simulink library "Linkage"  (R2025b)
settings: Solver=VariableStepAuto  StartTime=0.0  StopTime=10.0  RelTol=1e-3
undefined symbols (not defined in the file): Axle1D, AxleIn, Chassis, Init, RaceFix, RaceSpin, Vehicle, Visual, X, Y, Z
libraries: sm_lib x940, nesl_utility x136, fl_lib x6, Linkage_Systems x2, SteeringWheel x2, Linkage_Decoupled x2, AntiRollBar_Systems x1, Steer_Rack_None x1, Steer_Rack_WheelDrivenRack1UJoint x1
(part 25 of 25)

== system Linkage/Susp/Linkage Decoupled/Steer/Wheel Driven Rack 1UJoint/Driver/Human/Leg L/Toe L ==
  ReferenceFrame : sm_lib/Frames and Transforms/Reference Frame
  Solid : sm_lib/Body Elements/File Solid  ExtGeomFileName=Human_toe_L.STEP  UnitType=FromFile  ExtGeomFileUnits=m  StepReaderType=HEX  ExportConvexHullGeometry=off  InertiaType=CalculateFromGeometry  BasedOnType=Density  Density=rho_human  DensityUnits=kg/m^3  Mass=0  MassUnits=kg  CenterOfMass=[0 0 0]  CenterOfMassUnits=mm  MomentsOfInertia=[1 1 1]  MomentsOfInertiaUnits=kg*mm^2  ProductsOfInertia=[0 0 0]  ProductsOfInertiaUnits=kg*mm^2  GraphicType=FromGeometry  MarkerShape=Sphere  MarkerSize=10  GraphicVisPropType=SimpleVisualProperties  GraphicDiffuseColor=clr_human  GraphicOpacity=opc_human  GraphicSpecularColor=[0.5 0.5 0.5 1.0]  GraphicAmbientColor=[0.15 0.15 0.15 1.0]  GraphicEmissiveColor=[0.0 0.0 0.0 1.0]  GraphicShininess=75  DoExposeReferenceFrame=on  SerializedFrames=<Frames/>
  Transform : sm_lib/Frames and Transforms/Rigid Transform  RotationMethod=ArbitraryAxis  FollAlignAxisA=+X  BaseAlignAxisA=+Y  FollAlignAxisB=+Y  BaseAlignAxisB=+Z  RotationStandardAxis=+Z  RotationAngle=0.087266462599702  RotationAngleUnits=rad  RotationArbitraryAxis=[1 -4.97119394825472e-15 -1.1612709063123e-14]  RotationSequenceAxes=FollowerAxes  RotationSequence=XYX  RotationSequenceAngles=[0 0 0]  RotationSequenceAnglesUnits=deg  RotationMatrix=[1 0 0; 0 1 0; 0 0 1]  Quaternion=[1 0 0 0]  TranslationMethod=Cartesian  TranslationCartesianOffset=[-1.46549439250521e-14 -82.7975674566105 4.68055928693002]  TranslationCartesianOffsetUnits=mm  TranslationStandardAxis=+Z  TranslationStandardOffset=0  TranslationStandardOffsetUnits=mm  TranslationROffset=0  TranslationROffsetUnits=m  TranslationThetaOffset=0  TranslationThetaOffsetUnits=deg  TranslationZOffset=0  TranslationZOffsetUnits=m
  F : PMIOPort  Side=Left
  connections:
  Transform/RConn1 -- F/RConn1
  Transform/LConn1 -- ReferenceFrame/RConn1 -- Solid/RConn1

== system Linkage/Susp/Linkage Decoupled/Steer/Wheel Driven Rack 1UJoint/Driver/Human/Leg R/Foot R ==
  ReferenceFrame : sm_lib/Frames and Transforms/Reference Frame
  Solid : sm_lib/Body Elements/File Solid  ExtGeomFileName=Human_foot_R.STEP  UnitType=FromFile  ExtGeomFileUnits=m  StepReaderType=HEX  ExportConvexHullGeometry=off  InertiaType=CalculateFromGeometry  BasedOnType=Density  Density=rho_human  DensityUnits=kg/m^3  Mass=0  MassUnits=kg  CenterOfMass=[0 0 0]  CenterOfMassUnits=mm  MomentsOfInertia=[1 1 1]  MomentsOfInertiaUnits=kg*mm^2  ProductsOfInertia=[0 0 0]  ProductsOfInertiaUnits=kg*mm^2  GraphicType=FromGeometry  MarkerShape=Sphere  MarkerSize=10  GraphicVisPropType=SimpleVisualProperties  GraphicDiffuseColor=clr_human  GraphicOpacity=opc_human  GraphicSpecularColor=[0.5 0.5 0.5 1.0]  GraphicAmbientColor=[0.15 0.15 0.15 1.0]  GraphicEmissiveColor=[0.0 0.0 0.0 1.0]  GraphicShininess=75  DoExposeReferenceFrame=on  SerializedFrames=<Frames/>
  Transform : sm_lib/Frames and Transforms/Rigid Transform  RotationMethod=ArbitraryAxis  FollAlignAxisA=+X  BaseAlignAxisA=+Y  FollAlignAxisB=+Y  BaseAlignAxisB=+Z  RotationStandardAxis=+Z  RotationAngle=0  RotationAngleUnits=rad  RotationArbitraryAxis=[0 0 0]  RotationSequenceAxes=FollowerAxes  RotationSequence=XYX  RotationSequenceAngles=[0 0 0]  RotationSequenceAnglesUnits=deg  RotationMatrix=[1 0 0; 0 1 0; 0 0 1]  Quaternion=[1 0 0 0]  TranslationMethod=Cartesian  TranslationCartesianOffset=[0 0 0]  TranslationCartesianOffsetUnits=mm  TranslationStandardAxis=+Z  TranslationStandardOffset=0  TranslationStandardOffsetUnits=mm  TranslationROffset=0  TranslationROffsetUnits=m  TranslationThetaOffset=0  TranslationThetaOffsetUnits=deg  TranslationZOffset=0  TranslationZOffsetUnits=m
  Transform1 : sm_lib/Frames and Transforms/Rigid Transform  RotationMethod=ArbitraryAxis  FollAlignAxisA=+X  BaseAlignAxisA=+Y  FollAlignAxisB=+Y  BaseAlignAxisB=+Z  RotationStandardAxis=+Z  RotationAngle=2.0943951023932  RotationAngleUnits=rad  RotationArbitraryAxis=[0.577350269189626 0.577350269189626 0.577350269189626]  RotationSequenceAxes=FollowerAxes  RotationSequence=XYX  RotationSequenceAngles=[0 0 0]  RotationSequenceAnglesUnits=deg  RotationMatrix=[1 0 0; 0 1 0; 0 0 1]  Quaternion=[1 0 0 0]  TranslationMethod=Cartesian  TranslationCartesianOffset=[-90.2524899999995 -95.0000000000001 -945.84775686]  TranslationCartesianOffsetUnits=mm  TranslationStandardAxis=+Z  TranslationStandardOffset=0  TranslationStandardOffsetUnits=mm  TranslationROffset=0  TranslationROffsetUnits=m  TranslationThetaOffset=0  TranslationThetaOffsetUnits=deg  TranslationZOffset=0  TranslationZOffsetUnits=m
  F1 : PMIOPort  Side=Left
  F : PMIOPort  Port=2  Side=Left
  connections:
  Transform1/RConn1 -- F1/RConn1
  Transform/RConn1 -- F/RConn1
  Transform1/LConn1 -- ReferenceFrame/RConn1 -- Solid/RConn1 -- Transform/LConn1

== system Linkage/Susp/Linkage Decoupled/Steer/Wheel Driven Rack 1UJoint/Driver/Human/Leg R/Leg Lower R ==
  ReferenceFrame : sm_lib/Frames and Transforms/Reference Frame
  Solid : sm_lib/Body Elements/File Solid  ExtGeomFileName=Human_leg_lower_R.STEP  UnitType=FromFile  ExtGeomFileUnits=m  StepReaderType=HEX  ExportConvexHullGeometry=off  InertiaType=CalculateFromGeometry  BasedOnType=Density  Density=rho_human  DensityUnits=kg/m^3  Mass=0  MassUnits=kg  CenterOfMass=[0 0 0]  CenterOfMassUnits=mm  MomentsOfInertia=[1 1 1]  MomentsOfInertiaUnits=kg*mm^2  ProductsOfInertia=[0 0 0]  ProductsOfInertiaUnits=kg*mm^2  GraphicType=FromGeometry  MarkerShape=Sphere  MarkerSize=10  GraphicVisPropType=SimpleVisualProperties  GraphicDiffuseColor=clr_human  GraphicOpacity=opc_human  GraphicSpecularColor=[0.5 0.5 0.5 1.0]  GraphicAmbientColor=[0.15 0.15 0.15 1.0]  GraphicEmissiveColor=[0.0 0.0 0.0 1.0]  GraphicShininess=75  DoExposeReferenceFrame=on  SerializedFrames=<Frames/>
  Transform : sm_lib/Frames and Transforms/Rigid Transform  RotationMethod=ArbitraryAxis  FollAlignAxisA=+X  BaseAlignAxisA=+Y  FollAlignAxisB=+Y  BaseAlignAxisB=+Z  RotationStandardAxis=+Z  RotationAngle=1.81417419955097  RotationAngleUnits=rad  RotationArbitraryAxis=[0.440666253836566 0.7820655378287 0.440666253836566]  RotationSequenceAxes=FollowerAxes  RotationSequence=XYX  RotationSequenceAngles=[0 0 0]  RotationSequenceAnglesUnits=deg  RotationMatrix=[1 0 0; 0 1 0; 0 0 1]  Quaternion=[1 0 0 0]  TranslationMethod=Cartesian  TranslationCartesianOffset=[-90.2524948099997 6.94251895000275 -465.147514340017]  TranslationCartesianOffsetUnits=mm  TranslationStandardAxis=+Z  TranslationStandardOffset=0  TranslationStandardOffsetUnits=mm  TranslationROffset=0  TranslationROffsetUnits=m  TranslationThetaOffset=0  TranslationThetaOffsetUnits=deg  TranslationZOffset=0  TranslationZOffsetUnits=m
  Transform1 : sm_lib/Frames and Transforms/Rigid Transform  RotationMethod=ArbitraryAxis  FollAlignAxisA=+X  BaseAlignAxisA=+Y  FollAlignAxisB=+Y  BaseAlignAxisB=+Z  RotationStandardAxis=+Z  RotationAngle=0.168839148981579  RotationAngleUnits=rad  RotationArbitraryAxis=[1 -1.13358649593422e-14 -2.20648188183204e-15]  RotationSequenceAxes=FollowerAxes  RotationSequence=XYX  RotationSequenceAngles=[0 0 0]  RotationSequenceAnglesUnits=deg  RotationMatrix=[1 0 0; 0 1 0; 0 0 1]  Quaternion=[1 0 0 0]  TranslationMethod=Cartesian  TranslationCartesianOffset=[-4.80450753315154e-06 -161.530492970631 -21.0644735114674]  TranslationCartesianOffsetUnits=mm  TranslationStandardAxis=+Z  TranslationStandardOffset=0  TranslationStandardOffsetUnits=mm  TranslationROffset=0  TranslationROffsetUnits=m  TranslationThetaOffset=0  TranslationThetaOffsetUnits=deg  TranslationZOffset=0  TranslationZOffsetUnits=m
  F1 : PMIOPort  Side=Left
  F : PMIOPort  Port=2  Side=Left
  connections:
  Transform1/RConn1 -- F1/RConn1
  Transform/RConn1 -- F/RConn1
  Transform1/LConn1 -- Transform/LConn1 -- ReferenceFrame/RConn1 -- Solid/RConn1

== system Linkage/Susp/Linkage Decoupled/Steer/Wheel Driven Rack 1UJoint/Driver/Human/Leg R/Leg Upper R ==
  ReferenceFrame : sm_lib/Frames and Transforms/Reference Frame
  Solid : sm_lib/Body Elements/File Solid  ExtGeomFileName=Human_leg_upper_R.STEP  UnitType=FromFile  ExtGeomFileUnits=m  StepReaderType=HEX  ExportConvexHullGeometry=off  InertiaType=CalculateFromGeometry  BasedOnType=Density  Density=rho_human  DensityUnits=kg/m^3  Mass=0  MassUnits=kg  CenterOfMass=[0 0 0]  CenterOfMassUnits=mm  MomentsOfInertia=[1 1 1]  MomentsOfInertiaUnits=kg*mm^2  ProductsOfInertia=[0 0 0]  ProductsOfInertiaUnits=kg*mm^2  GraphicType=FromGeometry  MarkerShape=Sphere  MarkerSize=10  GraphicVisPropType=SimpleVisualProperties  GraphicDiffuseColor=clr_human  GraphicOpacity=opc_human  GraphicSpecularColor=[0.5 0.5 0.5 1.0]  GraphicAmbientColor=[0.15 0.15 0.15 1.0]  GraphicEmissiveColor=[0.0 0.0 0.0 1.0]  GraphicShininess=75  DoExposeReferenceFrame=on  SerializedFrames=<Frames/>
  Transform : sm_lib/Frames and Transforms/Rigid Transform  RotationMethod=ArbitraryAxis  FollAlignAxisA=+X  BaseAlignAxisA=+Y  FollAlignAxisB=+Y  BaseAlignAxisB=+Z  RotationStandardAxis=+Z  RotationAngle=2.0943951023932  RotationAngleUnits=rad  RotationArbitraryAxis=[0.577350269189626 0.577350269189626 0.577350269189626]  RotationSequenceAxes=FollowerAxes  RotationSequence=XYX  RotationSequenceAngles=[0 0 0]  RotationSequenceAnglesUnits=deg  RotationMatrix=[1 0 0; 0 1 0; 0 0 1]  Quaternion=[1 0 0 0]  TranslationMethod=Cartesian  TranslationCartesianOffset=[-90.2525043500121 6.94251895000207 -465.147514340004]  TranslationCartesianOffsetUnits=mm  TranslationStandardAxis=+Z  TranslationStandardOffset=0  TranslationStandardOffsetUnits=mm  TranslationROffset=0  TranslationROffsetUnits=m  TranslationThetaOffset=0  TranslationThetaOffsetUnits=deg  TranslationZOffset=0  TranslationZOffsetUnits=m
  Transform1 : sm_lib/Frames and Transforms/Rigid Transform  RotationMethod=ArbitraryAxis  FollAlignAxisA=+X  BaseAlignAxisA=+Y  FollAlignAxisB=+Y  BaseAlignAxisB=+Z  RotationStandardAxis=+Z  RotationAngle=0.675788058897533  RotationAngleUnits=rad  RotationArbitraryAxis=[0.998934159981039 0.0362097822206835 -0.0286250885502042]  RotationSequenceAxes=FollowerAxes  RotationSequence=XYX  RotationSequenceAngles=[0 0 0]  RotationSequenceAnglesUnits=deg  RotationMatrix=[1 0 0; 0 1 0; 0 0 1]  Quaternion=[1 0 0 0]  TranslationMethod=Cartesian  TranslationCartesianOffset=[-111.080007550003 1.18999978582224e-06 -27.7700042699978]  TranslationCartesianOffsetUnits=mm  TranslationStandardAxis=+Z  TranslationStandardOffset=0  TranslationStandardOffsetUnits=mm  TranslationROffset=0  TranslationROffsetUnits=m  TranslationThetaOffset=0  TranslationThetaOffsetUnits=deg  TranslationZOffset=0  TranslationZOffsetUnits=m
  F : PMIOPort  Side=Left
  F1 : PMIOPort  Port=2  Side=Left
  connections:
  Transform1/RConn1 -- F1/RConn1
  Transform/RConn1 -- F/RConn1
  Transform1/LConn1 -- Transform/LConn1 -- ReferenceFrame/RConn1 -- Solid/RConn1

== system Linkage/Susp/Linkage Decoupled/Steer/Wheel Driven Rack 1UJoint/Driver/Human/Leg R/Toe R ==
  ReferenceFrame : sm_lib/Frames and Transforms/Reference Frame
  Solid : sm_lib/Body Elements/File Solid  ExtGeomFileName=Human_toe_R.STEP  UnitType=FromFile  ExtGeomFileUnits=m  StepReaderType=HEX  ExportConvexHullGeometry=off  InertiaType=CalculateFromGeometry  BasedOnType=Density  Density=rho_human  DensityUnits=kg/m^3  Mass=0  MassUnits=kg  CenterOfMass=[0 0 0]  CenterOfMassUnits=mm  MomentsOfInertia=[1 1 1]  MomentsOfInertiaUnits=kg*mm^2  ProductsOfInertia=[0 0 0]  ProductsOfInertiaUnits=kg*mm^2  GraphicType=FromGeometry  MarkerShape=Sphere  MarkerSize=10  GraphicVisPropType=SimpleVisualProperties  GraphicDiffuseColor=clr_human  GraphicOpacity=opc_human  GraphicSpecularColor=[0.5 0.5 0.5 1.0]  GraphicAmbientColor=[0.15 0.15 0.15 1.0]  GraphicEmissiveColor=[0.0 0.0 0.0 1.0]  GraphicShininess=75  DoExposeReferenceFrame=on  SerializedFrames=<Frames/>
  Transform : sm_lib/Frames and Transforms/Rigid Transform  RotationMethod=ArbitraryAxis  FollAlignAxisA=+X  BaseAlignAxisA=+Y  FollAlignAxisB=+Y  BaseAlignAxisB=+Z  RotationStandardAxis=+Z  RotationAngle=2.14549020645537  RotationAngleUnits=rad  RotationArbitraryAxis=[0.593426057451643 0.543774795917203 0.593426057451644]  RotationSequenceAxes=FollowerAxes  RotationSequence=XYX  RotationSequenceAngles=[0 0 0]  RotationSequenceAnglesUnits=deg  RotationMatrix=[1 0 0; 0 1 0; 0 0 1]  Quaternion=[1 0 0 0]  TranslationMethod=Cartesian  TranslationCartesianOffset=[-90.252490000001 -95.0000000000059 -945.847756860017]  TranslationCartesianOffsetUnits=mm  TranslationStandardAxis=+Z  TranslationStandardOffset=0  TranslationStandardOffsetUnits=mm  TranslationROffset=0  TranslationROffsetUnits=m  TranslationThetaOffset=0  TranslationThetaOffsetUnits=deg  TranslationZOffset=0  TranslationZOffsetUnits=m
  F : PMIOPort  Side=Left
  connections:
  Transform/RConn1 -- F/RConn1
  Transform/LConn1 -- ReferenceFrame/RConn1 -- Solid/RConn1

== system Linkage/Susp/Linkage Decoupled/Steer/Rack Driven Shafts/Driver/Human/Body Sensor/Roll Pitch/Calculate aPitch ==
  Roll Angle : Inport
  uvec : Inport  Port=2
  Asin : Trigonometry  Operator=asin
  Cos : Trigonometry  Operator=cos
  Divide : Product  Inputs=*/
  Divide1 : Product  Inputs=*/
  Selector : Selector  InputPortWidth=3  IndexOptions=Index vector (dialog)  Indices=[3]  OutputSizes=1
  magnitude : Fcn  Expr=sqrt(u(1)*u(1)+u(2)*u(2)+u(3)*u(3))
  Angle : Outport  VectorParamsAs1DForOutWhenUnconnected=off
  wires:
  Cos/1 -> Divide/2
  Divide/1 -> Divide1/1
  Asin/1 -> Angle/1
  Roll Angle/1 -> Cos/1
  Selector/1 -> Divide/1
  magnitude/1 -> Divide1/2
  uvec/1 -> Selector/1, magnitude/1
  Divide1/1 -> Asin/1

== system Linkage/Susp/Linkage Decoupled/Steer/Rack Driven Shafts/Driver/Human/Body Sensor/Roll Pitch/Calculate aRoll ==
  uvec : Inport
  Demux : Demux  Outputs=3
  Mux : Mux  Inputs=2
  Trigonometric Function1 : Trigonometry  Operator=atan2
  magnitude : Fcn  Expr=sqrt(u(1)*u(1)+u(2)*u(2))
  Angle : Outport  VectorParamsAs1DForOutWhenUnconnected=off
  wires:
  Demux/1 -> Mux/1
  uvec/1 -> Demux/1
  Trigonometric Function1/1 -> Angle/1
  Demux/3 -> Trigonometric Function1/1
  Mux/1 -> magnitude/1
  magnitude/1 -> Trigonometric Function1/2
  Demux/2 -> Mux/2

== system Linkage/Susp/Linkage Decoupled/Steer/Rack Static Shafts/Driver/Human/Body Sensor/Roll Pitch/Calculate aPitch ==
  Roll Angle : Inport
  uvec : Inport  Port=2
  Asin : Trigonometry  Operator=asin
  Cos : Trigonometry  Operator=cos
  Divide : Product  Inputs=*/
  Divide1 : Product  Inputs=*/
  Selector : Selector  InputPortWidth=3  IndexOptions=Index vector (dialog)  Indices=[3]  OutputSizes=1
  magnitude : Fcn  Expr=sqrt(u(1)*u(1)+u(2)*u(2)+u(3)*u(3))
  Angle : Outport  VectorParamsAs1DForOutWhenUnconnected=off
  wires:
  Cos/1 -> Divide/2
  Divide/1 -> Divide1/1
  Asin/1 -> Angle/1
  Roll Angle/1 -> Cos/1
  Selector/1 -> Divide/1
  magnitude/1 -> Divide1/2
  uvec/1 -> Selector/1, magnitude/1
  Divide1/1 -> Asin/1

== system Linkage/Susp/Linkage Decoupled/Steer/Rack Static Shafts/Driver/Human/Body Sensor/Roll Pitch/Calculate aRoll ==
  uvec : Inport
  Demux : Demux  Outputs=3
  Mux : Mux  Inputs=2
  Trigonometric Function1 : Trigonometry  Operator=atan2
  magnitude : Fcn  Expr=sqrt(u(1)*u(1)+u(2)*u(2))
  Angle : Outport  VectorParamsAs1DForOutWhenUnconnected=off
  wires:
  Demux/1 -> Mux/1
  uvec/1 -> Demux/1
  Trigonometric Function1/1 -> Angle/1
  Demux/3 -> Trigonometric Function1/1
  Mux/1 -> magnitude/1
  magnitude/1 -> Trigonometric Function1/2
  Demux/2 -> Mux/2

== system Linkage/Susp/Linkage Decoupled/Steer/Rack Wheel/Driver/Human/Body Sensor/Roll Pitch/Calculate aPitch ==
  Roll Angle : Inport
  uvec : Inport  Port=2
  Asin : Trigonometry  Operator=asin
  Cos : Trigonometry  Operator=cos
  Divide : Product  Inputs=*/
  Divide1 : Product  Inputs=*/
  Selector : Selector  InputPortWidth=3  IndexOptions=Index vector (dialog)  Indices=[3]  OutputSizes=1
  magnitude : Fcn  Expr=sqrt(u(1)*u(1)+u(2)*u(2)+u(3)*u(3))
  Angle : Outport  VectorParamsAs1DForOutWhenUnconnected=off
  wires:
  Cos/1 -> Divide/2
  Divide/1 -> Divide1/1
  Asin/1 -> Angle/1
  Roll Angle/1 -> Cos/1
  Selector/1 -> Divide/1
  magnitude/1 -> Divide1/2
  uvec/1 -> Selector/1, magnitude/1
  Divide1/1 -> Asin/1

== system Linkage/Susp/Linkage Decoupled/Steer/Rack Wheel/Driver/Human/Body Sensor/Roll Pitch/Calculate aRoll ==
  uvec : Inport
  Demux : Demux  Outputs=3
  Mux : Mux  Inputs=2
  Trigonometric Function1 : Trigonometry  Operator=atan2
  magnitude : Fcn  Expr=sqrt(u(1)*u(1)+u(2)*u(2))
  Angle : Outport  VectorParamsAs1DForOutWhenUnconnected=off
  wires:
  Demux/1 -> Mux/1
  uvec/1 -> Demux/1
  Trigonometric Function1/1 -> Angle/1
  Demux/3 -> Trigonometric Function1/1
  Mux/1 -> magnitude/1
  magnitude/1 -> Trigonometric Function1/2
  Demux/2 -> Mux/2

== system Linkage/Susp/Linkage Decoupled/Steer/Wheel Driven Rack/Driver/Human/Body Sensor/Roll Pitch/Calculate aPitch ==
  Roll Angle : Inport
  uvec : Inport  Port=2
  Asin : Trigonometry  Operator=asin
  Cos : Trigonometry  Operator=cos
  Divide : Product  Inputs=*/
  Divide1 : Product  Inputs=*/
  Selector : Selector  InputPortWidth=3  IndexOptions=Index vector (dialog)  Indices=[3]  OutputSizes=1
  magnitude : Fcn  Expr=sqrt(u(1)*u(1)+u(2)*u(2)+u(3)*u(3))
  Angle : Outport  VectorParamsAs1DForOutWhenUnconnected=off
  wires:
  Cos/1 -> Divide/2
  Divide/1 -> Divide1/1
  Asin/1 -> Angle/1
  Roll Angle/1 -> Cos/1
  Selector/1 -> Divide/1
  magnitude/1 -> Divide1/2
  uvec/1 -> Selector/1, magnitude/1
  Divide1/1 -> Asin/1

== system Linkage/Susp/Linkage Decoupled/Steer/Wheel Driven Rack/Driver/Human/Body Sensor/Roll Pitch/Calculate aRoll ==
  uvec : Inport
  Demux : Demux  Outputs=3
  Mux : Mux  Inputs=2
  Trigonometric Function1 : Trigonometry  Operator=atan2
  magnitude : Fcn  Expr=sqrt(u(1)*u(1)+u(2)*u(2))
  Angle : Outport  VectorParamsAs1DForOutWhenUnconnected=off
  wires:
  Demux/1 -> Mux/1
  uvec/1 -> Demux/1
  Trigonometric Function1/1 -> Angle/1
  Demux/3 -> Trigonometric Function1/1
  Mux/1 -> magnitude/1
  magnitude/1 -> Trigonometric Function1/2
  Demux/2 -> Mux/2

== system Linkage/Susp/Linkage Decoupled/Steer/Wheel Driven Rack 1UJoint/Driver/Human/Body Sensor/Roll Pitch/Calculate aPitch ==
  Roll Angle : Inport
  uvec : Inport  Port=2
  Asin : Trigonometry  Operator=asin
  Cos : Trigonometry  Operator=cos
  Divide : Product  Inputs=*/
  Divide1 : Product  Inputs=*/
  Selector : Selector  InputPortWidth=3  IndexOptions=Index vector (dialog)  Indices=[3]  OutputSizes=1
  magnitude : Fcn  Expr=sqrt(u(1)*u(1)+u(2)*u(2)+u(3)*u(3))
  Angle : Outport  VectorParamsAs1DForOutWhenUnconnected=off
  wires:
  Cos/1 -> Divide/2
  Divide/1 -> Divide1/1
  Asin/1 -> Angle/1
  Roll Angle/1 -> Cos/1
  Selector/1 -> Divide/1
  magnitude/1 -> Divide1/2
  uvec/1 -> Selector/1, magnitude/1
  Divide1/1 -> Asin/1

== system Linkage/Susp/Linkage Decoupled/Steer/Wheel Driven Rack 1UJoint/Driver/Human/Body Sensor/Roll Pitch/Calculate aRoll ==
  uvec : Inport
  Demux : Demux  Outputs=3
  Mux : Mux  Inputs=2
  Trigonometric Function1 : Trigonometry  Operator=atan2
  magnitude : Fcn  Expr=sqrt(u(1)*u(1)+u(2)*u(2))
  Angle : Outport  VectorParamsAs1DForOutWhenUnconnected=off
  wires:
  Demux/1 -> Mux/1
  uvec/1 -> Demux/1
  Trigonometric Function1/1 -> Angle/1
  Demux/3 -> Trigonometric Function1/1
  Mux/1 -> magnitude/1
  magnitude/1 -> Trigonometric Function1/2
  Demux/2 -> Mux/2
